simulink model "Drone_simulation_PX4"  (R2025b)
settings: Solver=FixedStepAuto  StartTime=0.0  StopTime=inf  RelTol=1e-6
undefined symbols (not defined in the file): CommParams, fractalcoef, g, Gravity, HIL_GPS_Ts, HIL_HEARTBEAT_Ts, HIL_SENSOR_Ts, HIL_STATE_QUATERNION_Ts, IC, omega_max, Payload, PhysicalScaling, rho_0, SimParams, tau_motor, Tmax_total, Total_mass
libraries: uavmavlinklib x25, slrealtimeiplib x6, sim3dlib x4, aerolibatmos2 x2, matrix_library x1, simulink_extras x1, aerolibasang x1, sensorgpslib x1, mspsensorlib x1, sharedutil x1, aerolibconvert2 x1
(part 1 of 3)
settings Model: Creator=marku  LastModifiedBy=marku
settings SolverCC: AutoInsertRateTranBlk=on
settings OptimizationCC: DefaultParameterBehavior=Inlined  EnhancedBackFolding=on  PassReuseOutputArgsAs=Individual arguments  ZeroExternalMemoryAtStartup=off  ZeroInternalMemoryAtStartup=off  MaxStackSize=64  OptimizeBlockOrder=speed  DifferentSizesBufferReuse=on  OptimizationCustomize=off  EfficientTunableParamExpr=on
settings DebuggingCC: IntegerOverflowMsg=none  ParameterPrecisionLossMsg=none  ParameterTunabilityLossMsg=error  IntegerSaturationMsg=none
settings HardwareCC: ProdBitPerPointer=32.0  ProdBitPerSizeT=32.0  ProdBitPerPtrDiffT=32.0  ProdLargestAtomicInteger=Long  ProdLargestAtomicFloat=Double  ProdWordSize=32.0  ProdHWDeviceType=ARM Compatible->ARM Cortex
settings ModelReferenceCC: EnableParallelModelReferenceBuilds=on
settings SFSimCC: MATLABDynamicMemAlloc=off
settings RTWCC: SystemTargetFile=ert.tlc  TemplateMakefile=ert_default_tmf  Toolchain=GNU Tools for PX4 Autopilots  Description=Embedded Coder
settings CodeAppCC: ForceParamTrailComments=on  IgnoreCustomStorageClasses=off  OperatorAnnotations=on  SimulinkDataObjDesc=on  SFDataObjDesc=on  InsertBlockDesc=on
settings ERTTargetCC: ExtModeTransport=2.0  ExtModeStaticAlloc=on  ExtModeMexFile=ext_xcp  ExtModeIntrfLevel=Level2 - Open  InlinedParameterPlacement=Hierarchical  ERTCustomFileTemplate=example_file_process.tlc  SupportContinuousTime=on

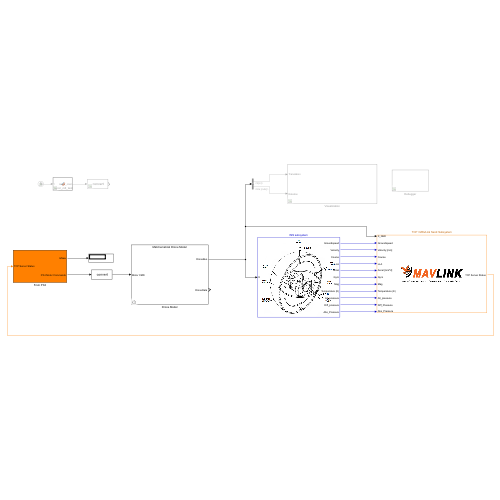
[thumbnail: Simulink's stored preview of the top-level diagram]
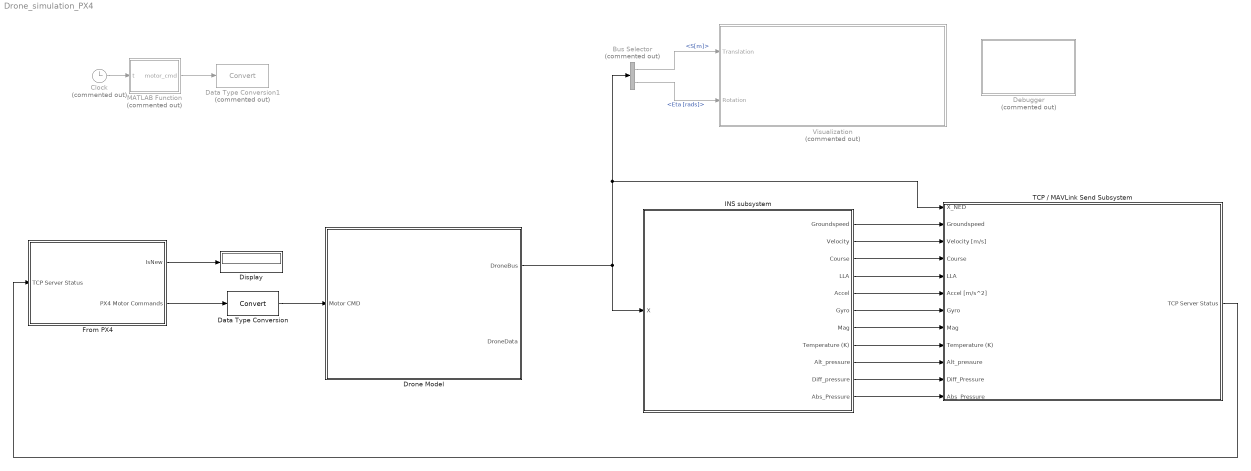
== system Drone_simulation_PX4 ==
  Bus Selector : BusSelector  Commented=on  OutputSignals=State.S[m],State.Eta [rads]
  Clock : Clock  Commented=on
  Data Type Conversion : DataTypeConversion  SaturateOnIntegerOverflow=off  RndMeth=Floor
  Data Type Conversion1 : DataTypeConversion  Commented=on  SaturateOnIntegerOverflow=off  RndMeth=Floor
  Debugger : Subsystem  Commented=on
  Display : Display
  Drone Model : Subsystem  Variant=on
  From PX4 : Subsystem
  INS subsystem : Subsystem
      mask Display: image('INS.png');
  MATLAB Function : MATLAB Function  Commented=on  TreatAsAtomicUnit=on
  TCP / MAVLink Send Subsystem : Subsystem
      mask Display: image('MavLink.png');
  Visualization : Subsystem  Commented=on
  wires:
  INS subsystem/10(Diff_pressure) -> TCP / MAVLink Send Subsystem/11(Diff_Pressure)
  INS subsystem/1(Groundspeed) -> TCP / MAVLink Send Subsystem/2(Groundspeed)
  INS subsystem/2(Velocity) -> TCP / MAVLink Send Subsystem/3(Velocity [m/s])
  INS subsystem/3(Course) -> TCP / MAVLink Send Subsystem/4(Course)
  INS subsystem/4(LLA) -> TCP / MAVLink Send Subsystem/5(LLA)
  INS subsystem/5(Accel) -> TCP / MAVLink Send Subsystem/6(Accel [m/s^2])
  INS subsystem/6(Gyro) -> TCP / MAVLink Send Subsystem/7(Gyro)
  INS subsystem/7(Mag) -> TCP / MAVLink Send Subsystem/8(Mag)
  INS subsystem/8(Temperature (K)) -> TCP / MAVLink Send Subsystem/9(Temperature (K))
  INS subsystem/9(Alt_pressure) -> TCP / MAVLink Send Subsystem/10(Alt_pressure)
  INS subsystem/11(Abs_Pressure) -> TCP / MAVLink Send Subsystem/12(Abs_Pressure)
  TCP / MAVLink Send Subsystem/1(TCP Server Status) -> From PX4/1(TCP Server Status)
  Bus Selector/1 -> Visualization/1(Translation)  "<S[m]>"
  Drone Model/1(DroneBus) -> Bus Selector/1, TCP / MAVLink Send Subsystem/1(X_NED), INS subsystem/1(X)
  Bus Selector/2 -> Visualization/2(Rotation)  "<Eta [rads]>"
  Clock/1 -> MATLAB Function/1(t)
  MATLAB Function/1(motor_cmd) -> Data Type Conversion1/1
  Data Type Conversion/1 -> Drone Model/1(Motor CMD)
  From PX4/2(PX4 Motor Commands) -> Data Type Conversion/1
  From PX4/1(IsNew) -> Display/1

== system Drone_simulation_PX4/Debugger ==
  Bus Creator : BusCreator  Inputs=6
  Clock : Clock
  Constant : Constant  Value=3
  Hover : Constant  Value=-Total_mass*Gravity
  MATLAB Function : MATLAB Function  TreatAsAtomicUnit=on
  MATLAB Function1 : MATLAB Function  TreatAsAtomicUnit=on
  MATLAB Function2 : MATLAB Function  TreatAsAtomicUnit=on
  Manual Switch : ManualSwitch  CurrentSetting=0
  TCP / MAVLink Send Subsystem1 : Subsystem
      mask Display: image('MavLink.png');
  wires:
  MATLAB Function/6(Orientation) -> Bus Creator/6
  MATLAB Function1/1(m) -> Manual Switch/1
  Clock/1 -> MATLAB Function1/1(t)
  MATLAB Function/5(Eta) -> Bus Creator/5
  Hover/1 -> MATLAB Function2/3(T_hover)
  MATLAB Function/2(S_dot) -> Bus Creator/2
  MATLAB Function/1(S) -> Bus Creator/1
  MATLAB Function/4(Omega) -> Bus Creator/4
  Constant/1 -> MATLAB Function1/2(test_id)
  MATLAB Function/3(S_ddot) -> Bus Creator/3

== system Drone_simulation_PX4/Drone Model ==
  Motor CMD : Inport
  Matchematical Drone Model : Subsystem  TreatAsAtomicUnit=on  VariantControl=Config.Plant.VariantValue == 1
  Simscape_Drone_Model : ModelReference  ModelNameDialog=Simscape_Drone_Model.slx  SimulationMode=Normal  VariantControl=Config.Plant.VariantValue == 2  ModelReferenceVersion=1.166
  DroneBus : Outport
  DroneData : Outport  Port=2

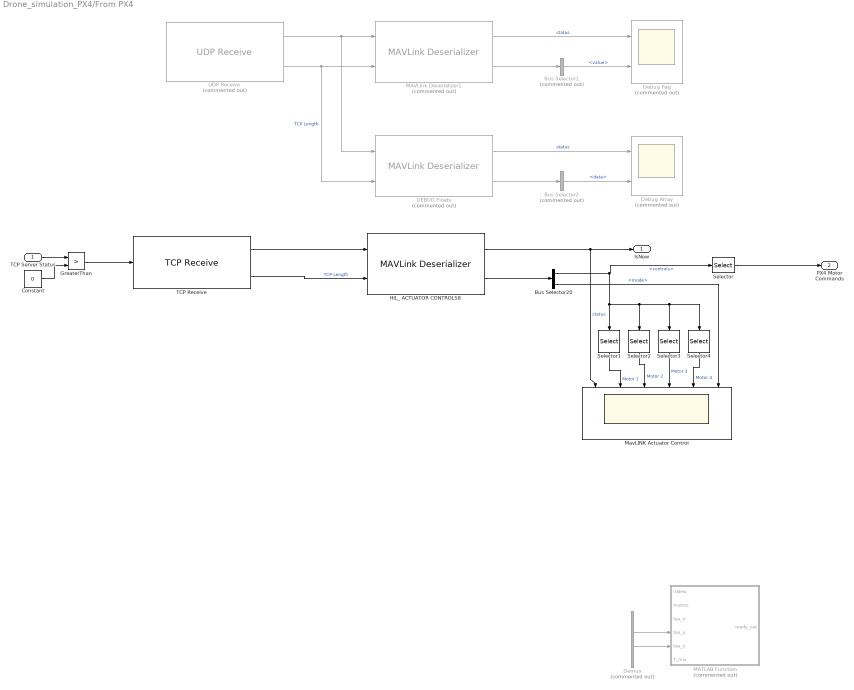
== system Drone_simulation_PX4/From PX4 ==
  TCP Server Status : Inport
  Bus Selector1 : BusSelector  Commented=on  OutputSignals=Payload.value
  Bus Selector2 : BusSelector  Commented=on  OutputSignals=Payload.data
  Bus Selector20 : BusSelector  OutputSignals=Payload.controls,Payload.mode
  Constant : Constant  Value=0  OutDataTypeStr=Inherit: Inherit via back propagation  SampleTime=-1
  DEBUG Floats : uavmavlinklib/MAVLink Deserializer  Commented=on  dialectSource=Select from standard MAVLink dialects  dialect=common.xml  dialectCustom=common.xml  version=2  messageType=DEBUG_FLOAT_ARRAY  inputDataLength=on  SystemIDFilter=off  systemID=1  ComponentIDFilter=off  componentID=1  queueMsg=off  queueMsgSize=50  dropNum=off
  Debug Array : Scope  Commented=on  NumInputPorts=2
      settings: ActiveDisplayYMinimum=-1  ActiveDisplayYMaximum=1  DataLoggingVariableName=ScopeData6
  Debug flag : Scope  Commented=on  NumInputPorts=2
      settings: ActiveDisplayYMinimum=-1  ActiveDisplayYMaximum=1  DataLoggingVariableName=ScopeData9
  Demux : Demux  Commented=on
  GreaterThan : RelationalOperator  Operator=>  OutDataTypeStr=Inherit: Inherit via back propagation  RndMeth=Simplest  InputSameDT=off
  HIL_ ACTUATOR CONTROLS8 : uavmavlinklib/MAVLink Deserializer  dialectSource=Select from standard MAVLink dialects  dialect=common.xml  dialectCustom=common.xml  version=2  messageType=HIL_ACTUATOR_CONTROLS  inputDataLength=on  SystemIDFilter=off  systemID=1  ComponentIDFilter=off  componentID=1  queueMsg=off  queueMsgSize=50  dropNum=off
  MATLAB Function : MATLAB Function  Commented=on  TreatAsAtomicUnit=on
  MAVLink Deserializer1 : uavmavlinklib/MAVLink Deserializer  Commented=on  dialectSource=Select from standard MAVLink dialects  dialect=common.xml  dialectCustom=common.xml  version=2  messageType=DEBUG  inputDataLength=on  SystemIDFilter=off  systemID=1  ComponentIDFilter=off  componentID=1  queueMsg=off  queueMsgSize=50  dropNum=off
  MavLINK Actuator Control : Scope  NumInputPorts=6
      settings: ActiveDisplayYMinimum=-0.12499999999999997  ActiveDisplayYMaximum=1.125  DataLoggingVariableName=ScopeData28
  Selector : Selector  InputPortWidth=16  IndexOptions=Index vector (dialog)  Indices=[1 2 3 4]  OutputSizes=1
  Selector1 : Selector  InputPortWidth=16  IndexOptions=Index vector (dialog)  Indices=[1]  OutputSizes=1
  Selector2 : Selector  InputPortWidth=16  IndexOptions=Index vector (dialog)  Indices=[2]  OutputSizes=1
  Selector3 : Selector  InputPortWidth=16  IndexOptions=Index vector (dialog)  Indices=[3]  OutputSizes=1
  Selector4 : Selector  InputPortWidth=16  IndexOptions=Index vector (dialog)  Indices=[4]  OutputSizes=1
  TCP Receive : slrealtimeiplib/TCP Receive  socketAddPortVal=Server: <Use host-target connection>:4560  rcvWidth=512  sampleTime=-1
  UDP Receive : slrealtimeiplib/UDP Receive  Commented=on  useHostTargetConn=on  ipAddress=0.0.0.0  localPort=14540  rcvWidth=512  rcvFmAny=on  fmAddress='10.10.10.10'  sampleTime=-1  enableMessage=off  maxPackets=1
  IsNew : Outport
  PX4 Motor Commands : Outport  Port=2
  wires:
  Bus Selector2/1 -> Debug Array/2  "<data>"
  HIL_ ACTUATOR CONTROLS8/1 -> MavLINK Actuator Control/1, IsNew/1  "status"
  UDP Receive/2 -> DEBUG Floats/2, MAVLink Deserializer1/2  "TCP Length"
  UDP Receive/1 -> DEBUG Floats/1, MAVLink Deserializer1/1
  Bus Selector20/1 -> Selector/1, Selector2/1, Selector3/1, Selector4/1, Selector1/1  "<controls>"
  Bus Selector1/1 -> Debug flag/2  "<value>"
  Bus Selector20/2 -> MavLINK Actuator Control/6  "<mode>"
  TCP Receive/1 -> HIL_ ACTUATOR CONTROLS8/1
  MAVLink Deserializer1/2 -> Bus Selector1/1
  DEBUG Floats/1 -> Debug Array/1  "status"
  MAVLink Deserializer1/1 -> Debug flag/1  "status"
  TCP Receive/2 -> HIL_ ACTUATOR CONTROLS8/2  "TCP Length"
  HIL_ ACTUATOR CONTROLS8/2 -> Bus Selector20/1
  DEBUG Floats/2 -> Bus Selector2/1
  Selector/1 -> PX4 Motor Commands/1
  TCP Server Status/1 -> GreaterThan/1
  Constant/1 -> GreaterThan/2
  GreaterThan/1 -> TCP Receive/1
  ? -> Demux/1
  Demux/2 -> MATLAB Function/4(tau_y)
  Demux/3 -> MATLAB Function/5(tau_z)
  Selector1/1 -> MavLINK Actuator Control/2  "Motor 1"
  Selector2/1 -> MavLINK Actuator Control/3  "Motor 2"
  Selector3/1 -> MavLINK Actuator Control/4  "Motor 3"
  Selector4/1 -> MavLINK Actuator Control/5  "Motor 4"

== system Drone_simulation_PX4/INS subsystem ==
  X : Inport
  INS : Subsystem
      mask Display: image('INS.png');
  INS Data : Scope  Commented=on  NumInputPorts=11
      settings: ActiveDisplayString=10  ActiveDisplayYMinimum=-1.5003434559985596  ActiveDisplayYMaximum=13.503091103987041  DataLoggingVariableName=ScopeData3
  Groundspeed : Outport
  Velocity : Outport  Port=2
  Course : Outport  Port=3
  LLA : Outport  Port=4
  Accel : Outport  Port=5
  Gyro : Outport  Port=6
  Mag : Outport  Port=7
  Temperature (K) : Outport  Port=8
  Alt_pressure : Outport  Port=9
  Diff_pressure : Outport  Port=10
  Abs_Pressure : Outport  Port=11
  wires:
  INS/3(Groundspeed) -> Groundspeed/1, INS Data/3  "Groundpseed"
  INS/5(Accel) -> Accel/1, INS Data/5  "Acceleration"
  INS/1(LLA) -> LLA/1, INS Data/1  "LLA"
  INS/2(Velocity) -> Velocity/1, INS Data/2  "Velocity"
  INS/4(Course) -> Course/1, INS Data/4  "Course"
  INS/6(Gyro) -> Gyro/1, INS Data/6  "Gyro"
  INS/7(Mag) -> Mag/1, INS Data/7  "Mag"
  INS/8(Temperature (K)) -> Temperature (K)/1, INS Data/8  "Temperature [K]"
  INS/9(Alt_Pressure) -> Alt_pressure/1, INS Data/9  "Alt_pressure"
  INS/10(Diff_Pressure) -> Diff_pressure/1, INS Data/10  "Diff_pressure"
  INS/11(Abs_Pressure) -> Abs_Pressure/1, INS Data/11  "Abs_pressure"
  X/1 -> INS/1(X)

== system Drone_simulation_PX4/TCP // MAVLink Send Subsystem ==
  note: TCP Server
  note: Mavlink
  X_NED : Inport
  Groundspeed : Inport  Port=2
  Velocity [m/s] : Inport  Port=3
  Course : Inport  Port=4
  LLA : Inport  Port=5
  Accel [m/s^2] : Inport  Port=6
  Gyro : Inport  Port=7
  Mag : Inport  Port=8
  Temperature (K) : Inport  Port=9
  Alt_pressure : Inport  Port=10
  Diff_Pressure : Inport  Port=11
  Abs_Pressure : Inport  Port=12
  MAVLink Message Setup : Subsystem
  TCP : Subsystem
  TCP Server Status : Outport
  wires:
  Course/1 -> MAVLink Message Setup/4(Course)
  Groundspeed/1 -> MAVLink Message Setup/2(Groundspeed)
  Velocity [m/s]/1 -> MAVLink Message Setup/3(Velocity [m/s])
  Gyro/1 -> MAVLink Message Setup/7(Gyro)
  MAVLink Message Setup/1(MavLink Message) -> TCP/1(MavLink Message)
  Mag/1 -> MAVLink Message Setup/8(Mag)
  LLA/1 -> MAVLink Message Setup/5(LLA)
  Temperature (K)/1 -> MAVLink Message Setup/9(Temperature (K))
  Accel [m/s^2]/1 -> MAVLink Message Setup/6(Accel [m/s^2])
  Alt_pressure/1 -> MAVLink Message Setup/10(Alt_pressure)
  Diff_Pressure/1 -> MAVLink Message Setup/11(Diff_Pressure)
  X_NED/1 -> MAVLink Message Setup/1(X_NED)
  Abs_Pressure/1 -> MAVLink Message Setup/12(Abs_Pressure)
  TCP/1(TCP Server Status) -> TCP Server Status/1

== system Drone_simulation_PX4/Visualization ==
  Translation : Inport
  Rotation : Inport  Port=2
  Camera : sim3dlib/Simulation 3D Actor  Priority=1  ActorName=Sim3dActor2  ParentName=Scene Origin  Operation=Create at setup  InitScriptText=|  SampleTime=-1  Translation=[0 0 0]  Rotation=[0 0 0]  Scale=[1 1 1]  InputsText=Sim3dActor2.Translation Sim3dActor2.Rotation  aMode=5  ActorTag=Sim3dActor2  ActorType=Sim3dActor  ID=2
      | % Reserved keywords:
      | % - Actor : handle to this actor object
      | % - World : handle to the world object
      | 
      | % Examples:
      | 
      | % Create a primitive geometry (optional)
      | % createShape(Actor, 'box', [1 1 1]);
      | 
      | % Initialize values (optional)
      | % Actor.Physics = true;
      | % Actor.Color = [1 0 0];
  Constant : Constant  Value=[0; 0; 0]
  Gain : Gain  Gain=[-1; -1; 1]
  Simulation 3D Actor : sim3dlib/Simulation 3D Actor  Priority=1  ActorName=Sim3dActor1  ParentName=Scene Origin  Operation=Create at setup  InitScriptText=|  SampleTime=-1  Translation=[0 0 0]  Rotation=[0 0 0]  Scale=[1 1 1]  InputsText=Sim3dActor1.Translation Sim3dActor1.Rotation  aMode=5  ActorTag=Sim3dActor1  ActorType=Sim3dActor  ID=1
      | % Generic body shape for the 3D view (unit drone: 0.5 m across the rotors).
      | createShape(Actor, 'box', [0.5 0.5 0.1]);
  Simulation 3D Scene Configuration : sim3dlib/Simulation 3D Scene Configuration  Priority=0  ProjectFormat=Default Scenes  SceneDesc=Open surface  ProjectName=C:\Program Files\MATLAB\R2025b\toolbox\shared\sim3d_projects\automotive_project_windows\UE\WindowsNoEditor\VehicleSimulation.exe  ScenePath=/Game/Maps/HwStrght  EnableOpenDRIVE=off  vehTagList={'Custom';'Scene Origin';'Sim3dActor1';'Sim3dActor2'}  vehTag=Sim3dActor2  AttachedCameraRelativeTranslation=[-3 -3 2]  FreeCameraDefaultInitialTranslation=[-6, 0, 2]  AttachedCameraRelativeRotation=[-0 -20 45]  FreeCameraDefaultInitialRotation=[0, -15, 0]  ViewpointName=Custom  FreeCameraInitialTranslation=[-4 -4 2]  ViewpointTranslation=[0 0 0]  FreeCameraInitialRotation=[0 -15 45]  ViewpointRotation=[0 0 0]  OpVisEn=off  Ts=0.02  EnableWindow=off  EnableRemoteAccess=off  EnableWeather=off  SunAzimuth=90  SunAltitude=40.0  EnableGeospatialSun=off  Latitude=0  Longitude=0  Date=2023-01-01  Time=10:30:00  GeoTimeZone=-5.0  SunDaylightSaving=off  wind=1  clouds=10  EnableVolumetricClouds=off  CloudCoverage=0  CloudAltitude=6  fog=0  rain=0  RaindropsEffect=off  SnowDensity=0  EnableGeospatial=off  TilesetSource=Earth terrain  UseTrueOrigin=off  OriginHeight=200  OriginLatitude=40.744652  OriginLongitude=-73.988864  MapStyle=Aerial  AdditionalAssetIDs=[]  UseAdvancedSunSky=off  SolarTime=11  TimeZone=-5  Day=21  Month=9  Year=2022  UseDaylightSavingTime=on  DSTStartDay=10  DSTStartMonth=3  DSTEndDay=3  DSTEndMonth=11  DSTSwitchHour=2  sensorTag=MainCamera1  sensorId=1  sensorName=MainCamera1  mountLoc=Origin  offsetFlag=off  tmountOffset=[0, 0, 0]  rmountOffset=[0, 0, 0]  HorizontalResolution=1280  VerticalResolution=720  HorizontalFOV=60  mountPoint=[0 0 0]  mountOrientation=[0 0 0]  aMode=0  ID=1  GeoTrigger=Inactive  ViewNameList={'Custom'}  ViewTranslationList={'[-4 -4 2]'}  ViewRotationList={'[0 -15 45]'}
      settings: LibrarySourceBlock=aerolibsim3d/Simulation 3D Scene Configuration
  Simulation 3D Video Writer : sim3dlib/Simulation 3D Video Writer  Priority=1  Commented=on  Filename=PX4_square_flight.mp4  FileAction=Overwrite  Interval=[0 inf]  aMode=5
      settings: LibrarySourceBlock=sl3dlib/Simulation 3D/Utilities/Simulation 3D Video Writer
  Terminator : Terminator
  Terminator1 : Terminator
  Transpose : Math  Operator=transpose
  Transpose1 : Math  Operator=transpose
  Transpose2 : Math  Operator=transpose
  wires:
  Transpose/1 -> Camera/1, Simulation 3D Actor/1
  Simulation 3D Actor/1 -> Terminator/1
  Translation/1 -> Transpose/1
  Transpose1/1 -> Simulation 3D Actor/2
  Rotation/1 -> Gain/1
  Constant/1 -> Transpose2/1
  Transpose2/1 -> Camera/2
  Camera/1 -> Terminator1/1
  Gain/1 -> Transpose1/1

== system Drone_simulation_PX4/Debugger/TCP // MAVLink Send Subsystem1 ==
  note: MAVLink Message Setup
  note: TCP Server
  note: Mavlink
  note: Collected Signals
  note: MavLink signal setup
  HIL HEARTBEAT : Subsystem
  HIL STATE QUATERNION : Subsystem  Commented=on
  HIL_GPS : Subsystem
  HIL_SENSOR : Subsystem
  MAVLink Concatenate : Concatenate  NumInputs=4
  Signal Debugging : Subsystem
  TCP : Subsystem
  TCP Server Status : Outport
  wires:
  [A4] -> MAVLink Concatenate/4
  HIL HEARTBEAT/1(HEARTBEAT_DATA) -> [A4]
  [A3] -> MAVLink Concatenate/2
  [A2] -> MAVLink Concatenate/3
  [A1] -> MAVLink Concatenate/1
  MAVLink Concatenate/1 -> TCP/1(MavLink Message)  "MavLink Message"
  HIL STATE QUATERNION/1(HIL_STATE_QUATERNION_bytes) -> [A3], Signal Debugging/1(HIL_STATE_QUATERNION_bytes)
  HIL_SENSOR/1(HIL_SENSOR_bytes) -> Signal Debugging/3(HIL_SENSOR_bytes), [A1]
  HIL_GPS/1(HIL_SENSOR_bytes) -> Signal Debugging/2(HIL_GPS_bytes), [A2]
  TCP/1(TCP Server Status) -> TCP Server Status/1

== system Drone_simulation_PX4/Drone Model/Matchematical Drone Model ==
  Motor CMD : Inport
  Constant : Constant  Value=0
  Drone Dynamics : Subsystem
      mask Display: disp('Mechanical System')
  ENU to NED : Subsystem
      mask Display: image('World Frame Conversion.png');
  Hover : Constant  Commented=on  Value=single(sqrt(Total_mass*g/Tmax_total) * ones(4,1))
  MATLAB Function3 : MATLAB Function  Commented=on  TreatAsAtomicUnit=on
  Out Bus Element1 : Outport  PortName=DroneData  Element=Data
  Out Bus Element : Outport  Port=2  PortName=DroneBus  Element=State
  wires:
  Hover/1 -> MATLAB Function3/3(u_hover_cmd)
  Drone Dynamics/1(Drone_ENU) -> ENU to NED/1(Drone_ENU)
  Constant/1 -> Out Bus Element1/1
  ENU to NED/1(X_NED) -> Out Bus Element/1
  Motor CMD/1 -> Drone Dynamics/1(Inputs), MATLAB Function3/2(m_px4)

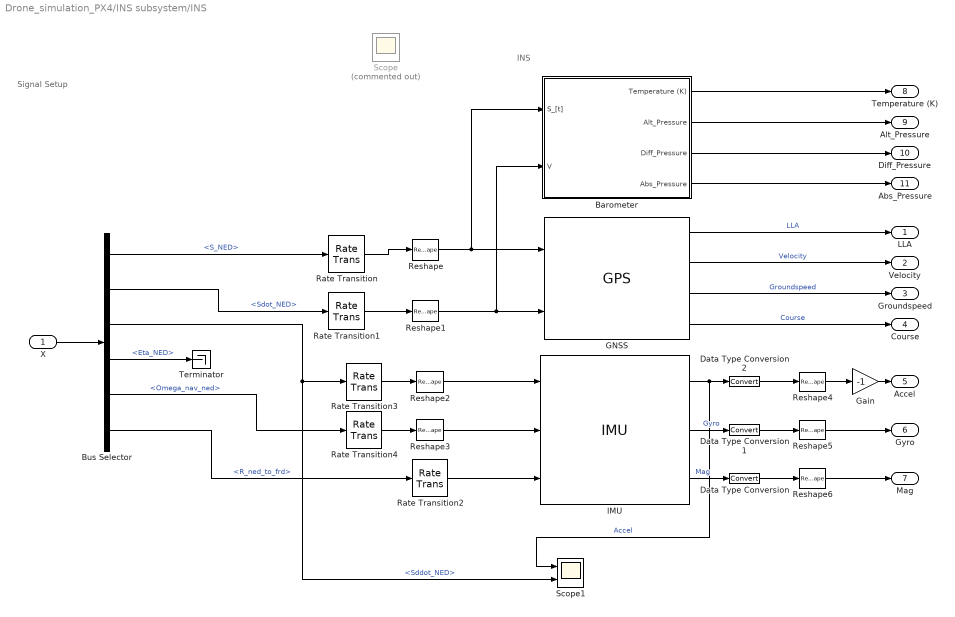
== system Drone_simulation_PX4/INS subsystem/INS ==
  note: INS
  note: Signal Setup
  X : Inport
  Barometer : Subsystem
  Bus Selector : BusSelector  OutputSignals=State.S_NED,State.Sdot_NED,State.Sddot_NED,State.Eta_NED,State.Omega_nav_ned,State.R_ned_to_frd
  Data Type Conversion : DataTypeConversion  SaturateOnIntegerOverflow=off  RndMeth=Floor
  Data Type Conversion1 : DataTypeConversion  SaturateOnIntegerOverflow=off  RndMeth=Floor
  Data Type Conversion2 : DataTypeConversion  SaturateOnIntegerOverflow=off  RndMeth=Floor
  GNSS : sensorgpslib/GPS  DispRefFrame=NED  PositionInputFormat=Local  ReferenceLocation=SimParams.HomeLLA  HorizontalPositionAccuracy=0.001  VerticalPositionAccuracy=0.001  VelocityAccuracy=0.001  DecayFactor=0  SeedDouble=0  SimulateUsing=Code generation
      settings: LibrarySourceBlock=mspsensorlib/GPS
  Gain : Gain  Gain=-1  OutDataTypeStr=Inherit: Inherit via back propagation
  IMU : mspsensorlib/IMU  DispRefFrame=NED  TemperaturePort=off  Temperature=15  MagneticFieldPort=off  MagneticFieldNED=SimParams.MagneticFieldNED  MagneticFieldENU=[ -2.4169, 27.5550, 16.0849 ]  SeedDouble=0  SimulateUsing=Code generation  AccelParamsMeasurementRange=Inf  AccelParamsResolution=0  AccelParamsConstantBias=[ 0, 0, 0 ]  AccelParamsAxesMisalignment=[ 100, 0, 0; 0, 100, 0; 0, 0, 100 ]  AccelParamsNoiseDensity=[ 0, 0, 0 ]  AccelParamsBiasInstability=[ 0, 0, 0 ]  AccelParamsBiasInstabilityNumerator=fractalcoef().Numerator  AccelParamsBiasInstabilityDenominator=fractalcoef().Denominator  AccelParamsRandomWalk=[ 0, 0, 0 ]  AccelParamsNoiseType=double-sided  AccelParamsTemperatureBias=[ 0, 0, 0 ]  AccelParamsTemperatureScaleFactor=[ 0, 0, 0 ]  GyroParamsMeasurementRange=Inf  GyroParamsResolution=0  GyroParamsConstantBias=[ 0, 0, 0 ]  GyroParamsAxesMisalignment=[ 100, 0, 0; 0, 100, 0; 0, 0, 100 ]  GyroParamsAccelerationBias=[ 0, 0, 0 ]  GyroParamsNoiseDensity=[ 0, 0, 0 ]  GyroParamsBiasInstability=[ 0, 0, 0 ]  GyroParamsBiasInstabilityNumerator=fractalcoef().Numerator  GyroParamsBiasInstabilityDenominator=fractalcoef().Denominator  GyroParamsRandomWalk=[ 0, 0, 0 ]  GyroParamsNoiseType=double-sided  GyroParamsTemperatureBias=[ 0, 0, 0 ]  GyroParamsTemperatureScaleFactor=[ 0, 0, 0 ]  MagParamsMeasurementRange=Inf  MagParamsResolution=0  MagParamsConstantBias=[ 0, 0, 0 ]  MagParamsAxesMisalignment=[ 100, 0, 0; 0, 100, 0; 0, 0, 100 ]  MagParamsNoiseDensity=[ 0, 0, 0 ]  MagParamsBiasInstability=[ 0, 0, 0 ]  MagParamsBiasInstabilityNumerator=fractalcoef().Numerator  MagParamsBiasInstabilityDenominator=fractalcoef().Denominator  MagParamsRandomWalk=[ 0, 0, 0 ]  MagParamsNoiseType=double-sided  MagParamsTemperatureBias=[ 0, 0, 0 ]  MagParamsTemperatureScaleFactor=[ 0, 0, 0 ]
  Rate Transition{,1..4} (5 alike) : RateTransition  OutPortSampleTime=CommParams.INS.Ts
  Reshape : Reshape  OutputDimensionality=Customize  OutputDimensions=[1,3]
  Reshape1 : Reshape  OutputDimensionality=Customize  OutputDimensions=[1,3]
  Reshape2 : Reshape  OutputDimensionality=Row vector (2-D)
  Reshape3 : Reshape  OutputDimensionality=Row vector (2-D)
  Reshape4 : Reshape
  Reshape5 : Reshape
  Reshape6 : Reshape
  Scope : Scope  Commented=on
      settings: ActiveDisplayYMinimum=-1  ActiveDisplayYMaximum=1  DataLoggingVariableName=ScopeData10
  Scope1 : Scope  NumInputPorts=2
      settings: ActiveDisplayYMinimum=-8.196879445424031  ActiveDisplayYMaximum=18.133560919726278  DataLoggingVariableName=ScopeData15
  Terminator : Terminator
  LLA : Outport
  Velocity : Outport  Port=2
  Groundspeed : Outport  Port=3
  Course : Outport  Port=4
  Accel : Outport  Port=5
  Gyro : Outport  Port=6
  Mag : Outport  Port=7
  Temperature (K) : Outport  Port=8
  Alt_Pressure : Outport  Port=9
  Diff_Pressure : Outport  Port=10
  Abs_Pressure : Outport  Port=11
  wires:
  GNSS/4 -> Course/1  "Course"
  GNSS/1 -> LLA/1  "LLA"
  GNSS/2 -> Velocity/1  "Velocity"
  GNSS/3 -> Groundspeed/1  "Groundspeed"
  Rate Transition2/1 -> IMU/3
  IMU/2 -> Data Type Conversion1/1  "Gyro"
  IMU/3 -> Data Type Conversion/1  "Mag"
  Rate Transition/1 -> Reshape/1
  Rate Transition1/1 -> Reshape1/1
  Rate Transition3/1 -> Reshape2/1
  Rate Transition4/1 -> Reshape3/1
  Barometer/1(Temperature (K)) -> Temperature (K)/1
  Barometer/2(Alt_Pressure) -> Alt_Pressure/1
  Barometer/3(Diff_Pressure) -> Diff_Pressure/1
  Barometer/4(Abs_Pressure) -> Abs_Pressure/1
  IMU/1 -> Scope1/1, Data Type Conversion2/1  "Accel"
  Reshape4/1 -> Gain/1
  Reshape5/1 -> Gyro/1
  Reshape6/1 -> Mag/1
  Data Type Conversion/1 -> Reshape6/1
  Data Type Conversion1/1 -> Reshape5/1
  Data Type Conversion2/1 -> Reshape4/1
  Gain/1 -> Accel/1
  X/1 -> Bus Selector/1
  Bus Selector/1 -> Rate Transition/1  "<S_NED>"
  Bus Selector/2 -> Rate Transition1/1  "<Sdot_NED>"
  Bus Selector/3 -> Rate Transition3/1, Scope1/2  "<Sddot_NED>"
  Bus Selector/4 -> Terminator/1  "<Eta_NED>"
  Bus Selector/6 -> Rate Transition2/1  "<R_ned_to_frd>"
  Reshape/1 -> Barometer/1(S_[t]), GNSS/1
  Reshape1/1 -> Barometer/2(V), GNSS/2
  Reshape2/1 -> IMU/1
  Reshape3/1 -> IMU/2
  Bus Selector/5 -> Rate Transition4/1  "<Omega_nav_ned>"

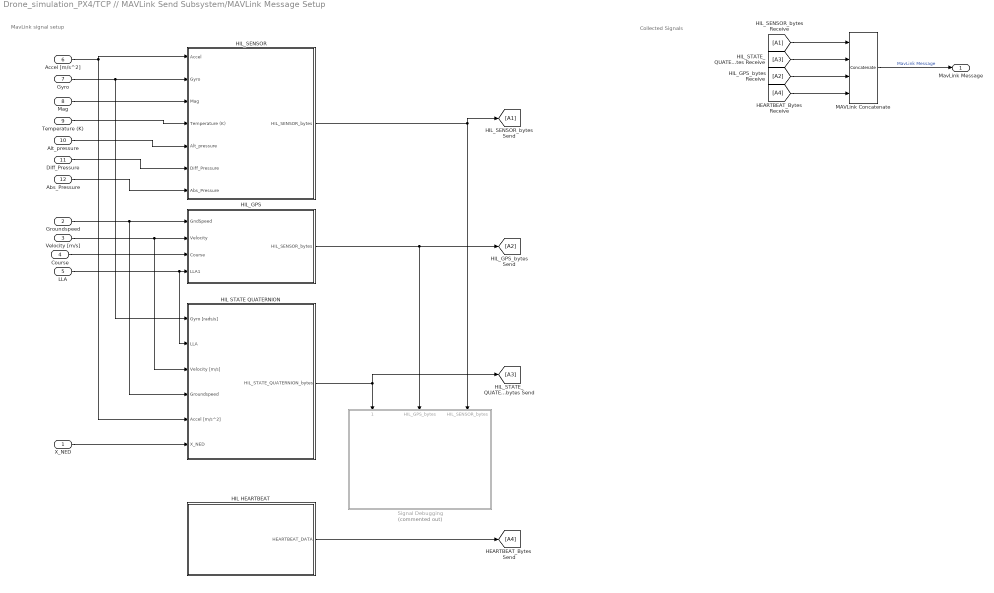
== system Drone_simulation_PX4/TCP // MAVLink Send Subsystem/MAVLink Message Setup ==
  note: MavLink signal setup
  note: Collected Signals
  X_NED : Inport
  Groundspeed : Inport  Port=2
  Velocity [m/s] : Inport  Port=3
  Course : Inport  Port=4
  LLA : Inport  Port=5
  Accel [m/s^2] : Inport  Port=6
  Gyro : Inport  Port=7
  Mag : Inport  Port=8
  Temperature (K) : Inport  Port=9
  Alt_pressure : Inport  Port=10
  Diff_Pressure : Inport  Port=11
  Abs_Pressure : Inport  Port=12
  HIL HEARTBEAT : Subsystem
  HIL STATE QUATERNION : Subsystem
  HIL_GPS : Subsystem
  HIL_SENSOR : Subsystem
  MAVLink Concatenate : Concatenate  NumInputs=4
  Signal Debugging : Subsystem  Commented=on
  MavLink Message : Outport
  wires:
  Alt_pressure/1 -> HIL_SENSOR/5(Alt_pressure)
  Mag/1 -> HIL_SENSOR/3(Mag)
  Diff_Pressure/1 -> HIL_SENSOR/6(Diff_Pressure)
  Temperature (K)/1 -> HIL_SENSOR/4(Temperature (K))
  Gyro/1 -> HIL STATE QUATERNION/1(Gyro [rads/s]), HIL_SENSOR/2(Gyro)
  HIL_GPS/1(HIL_SENSOR_bytes) -> Signal Debugging/2(HIL_GPS_bytes), [A2]
  Accel [m/s^2]/1 -> HIL STATE QUATERNION/5(Accel [m/s^2]), HIL_SENSOR/1(Accel)
  Abs_Pressure/1 -> HIL_SENSOR/7(Abs_Pressure)
  Course/1 -> HIL_GPS/3(Course)
  Velocity [m/s]/1 -> HIL STATE QUATERNION/3(Velocity [m/s]), HIL_GPS/2(Velocity)
  Groundspeed/1 -> HIL STATE QUATERNION/4(Groundspeed), HIL_GPS/1(GndSpeed)
  LLA/1 -> HIL STATE QUATERNION/2(LLA), HIL_GPS/4(LLA1)
  X_NED/1 -> HIL STATE QUATERNION/6(X_NED)
  HIL_SENSOR/1(HIL_SENSOR_bytes) -> Signal Debugging/3(HIL_SENSOR_bytes), [A1]
  HIL STATE QUATERNION/1(HIL_STATE_QUATERNION_bytes) -> [A3], Signal Debugging/1(HIL_STATE_QUATERNION_bytes)
  MAVLink Concatenate/1 -> MavLink Message/1  "MavLink Message"
  [A1] -> MAVLink Concatenate/1
  [A2] -> MAVLink Concatenate/3
  [A3] -> MAVLink Concatenate/2
  HIL HEARTBEAT/1(HEARTBEAT_DATA) -> [A4]
  [A4] -> MAVLink Concatenate/4

== system Drone_simulation_PX4/TCP // MAVLink Send Subsystem/TCP ==
  note: Server setup
  MavLink Message : Inport
  Boolean : Constant  OutDataTypeStr=Inherit: Inherit via back propagation  SampleTime=-1
  Display2 : Display
  Display3 : Display
  Reshape : Reshape
  TCP Send : slrealtimeiplib/TCP Send  socketAddPortVal=Server: <Use host-target connection>:4560  sampleTime=CommParams.HIL.Ts
  TCP Server : slrealtimeiplib/TCP Server  Priority=-1  useHostTargetConn=on  serverAddress=172.29.112.1  serverPort=4560  useNaglesAlgorithm=on
  Width : Width
  TCP Server Status : Outport
  wires:
  MavLink Message/1 -> Reshape/1
  TCP Server/1 -> TCP Server Status/1, Display2/1
  Boolean/1 -> TCP Server/1, TCP Send/1
  Reshape/1 -> TCP Send/2, Width/1
  TCP Send/1 -> Display3/1
  Width/1 -> TCP Send/3

== system Drone_simulation_PX4/Debugger/TCP // MAVLink Send Subsystem1/HIL HEARTBEAT ==
  Bus Assignment : BusAssignment  AssignedSignals=Payload.custom_mode,Payload.type,Payload.autopilot,Payload.base_mode,Payload.system_status,Payload.mavlink_version
  Constant : Constant  Value=0  OutDataTypeStr=Inherit: Inherit via back propagation  SampleTime=HIL_HEARTBEAT_Ts
  Constant1 : Constant  Value=2  OutDataTypeStr=Inherit: Inherit via back propagation  SampleTime=HIL_HEARTBEAT_Ts
  Constant2 : Constant  Value=8  OutDataTypeStr=Inherit: Inherit via back propagation  SampleTime=HIL_HEARTBEAT_Ts
  Constant3 : Constant  Value=0  OutDataTypeStr=Inherit: Inherit via back propagation  SampleTime=HIL_HEARTBEAT_Ts
  Constant4 : Constant  Value=4  OutDataTypeStr=Inherit: Inherit via back propagation  SampleTime=HIL_HEARTBEAT_Ts
  Constant5 : Constant  Value=3  OutDataTypeStr=Inherit: Inherit via back propagation  SampleTime=HIL_HEARTBEAT_Ts
  MAVLink Blank Message : uavmavlinklib/MAVLink Blank Message  dialectSource=Select from standard MAVLink dialects  dialect=common.xml  dialectCustom=common.xml  version=2  messageType=HEARTBEAT  SystemID=2  ComponentID=51  SampleTime=HIL_HEARTBEAT_Ts
  MAVLink Serializer : uavmavlinklib/MAVLink Serializer  dialectSource=Select from standard MAVLink dialects  dialect=common.xml  dialectCustom=common.xml  version=2  messageType=HEARTBEAT
  Rate Transition : RateTransition  OutPortSampleTime=HIL_HEARTBEAT_Ts
  Terminator : Terminator
  HEARTBEAT_DATA : Outport
  wires:
  Constant4/1 -> Bus Assignment/6
  Constant2/1 -> Bus Assignment/4
  MAVLink Blank Message/1 -> Bus Assignment/1
  Constant3/1 -> Bus Assignment/5
  Constant1/1 -> Bus Assignment/3
  Constant/1 -> Bus Assignment/2
  Constant5/1 -> Bus Assignment/7
  Bus Assignment/1 -> Rate Transition/1
  Rate Transition/1 -> MAVLink Serializer/1
  MAVLink Serializer/1 -> HEARTBEAT_DATA/1
  MAVLink Serializer/2 -> Terminator/1

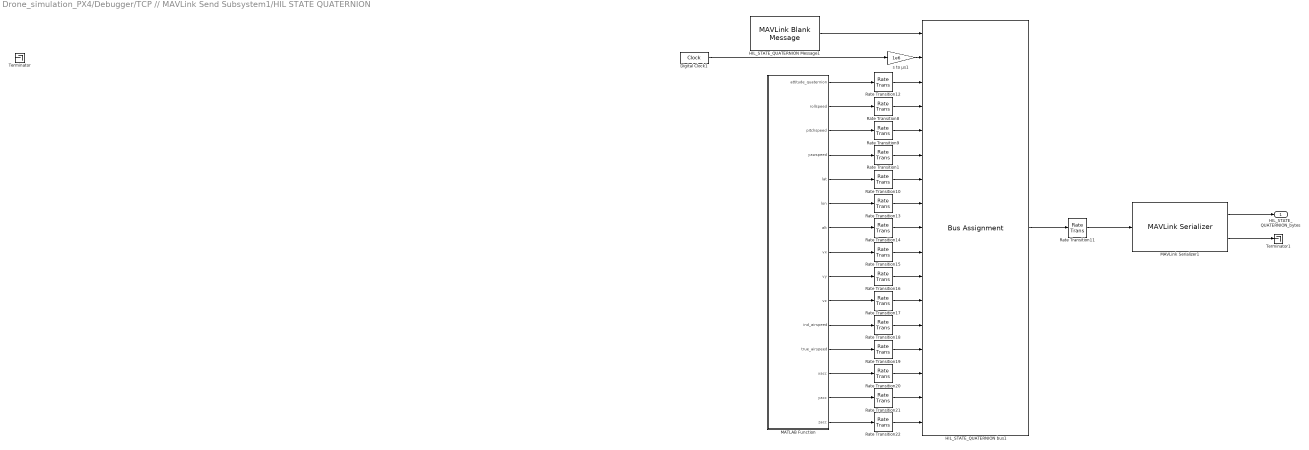
== system Drone_simulation_PX4/Debugger/TCP // MAVLink Send Subsystem1/HIL STATE QUATERNION ==
  Digital Clock1 : DigitalClock  SampleTime=HIL_STATE_QUATERNION_Ts
  HIL_STATE_QUATERNION Message1 : uavmavlinklib/MAVLink Blank Message  dialectSource=Select from standard MAVLink dialects  dialect=common.xml  dialectCustom=common.xml  version=2  messageType=HIL_STATE_QUATERNION  SystemID=2  ComponentID=51  SampleTime=-1
  HIL_STATE_QUATERNION bus1 : BusAssignment  AssignedSignals=Payload.time_usec,Payload.attitude_quaternion,Payload.rollspeed,Payload.pitchspeed,Payload.yawspeed,Payload.lat,Payload.lon,Payload.alt,Payload.vx,Payload.vy,Payload.vz,Payload.ind_airspeed,Payload.true_airspeed,Payload.xacc,Payload.yacc,Payload.zacc
  MATLAB Function : MATLAB Function  TreatAsAtomicUnit=on
  MAVLink Serializer1 : uavmavlinklib/MAVLink Serializer  dialectSource=Select from standard MAVLink dialects  dialect=common.xml  dialectCustom=common.xml  version=2  messageType=HIL_STATE_QUATERNION
  Rate Transition{1,8..22} (16 alike) : RateTransition  OutPortSampleTime=HIL_STATE_QUATERNION_Ts
  Terminator : Terminator
  Terminator1 : Terminator
  s to µs1 : Gain  Gain=1e6  OutDataTypeStr=uint64
  HIL_STATE_QUATERNION_bytes : Outport
  wires:
  Rate Transition11/1 -> MAVLink Serializer1/1
  HIL_STATE_QUATERNION bus1/1 -> Rate Transition11/1
  MAVLink Serializer1/2 -> Terminator1/1
  MAVLink Serializer1/1 -> HIL_STATE_QUATERNION_bytes/1
  HIL_STATE_QUATERNION Message1/1 -> HIL_STATE_QUATERNION bus1/1
  s to µs1/1 -> HIL_STATE_QUATERNION bus1/2
  Digital Clock1/1 -> s to µs1/1
  Rate Transition22/1 -> HIL_STATE_QUATERNION bus1/17
  Rate Transition21/1 -> HIL_STATE_QUATERNION bus1/16
  Rate Transition20/1 -> HIL_STATE_QUATERNION bus1/15
  Rate Transition19/1 -> HIL_STATE_QUATERNION bus1/14
  Rate Transition18/1 -> HIL_STATE_QUATERNION bus1/13
  Rate Transition12/1 -> HIL_STATE_QUATERNION bus1/3
  Rate Transition8/1 -> HIL_STATE_QUATERNION bus1/4
  Rate Transition9/1 -> HIL_STATE_QUATERNION bus1/5
  Rate Transition1/1 -> HIL_STATE_QUATERNION bus1/6
  Rate Transition10/1 -> HIL_STATE_QUATERNION bus1/7
  Rate Transition13/1 -> HIL_STATE_QUATERNION bus1/8
  Rate Transition14/1 -> HIL_STATE_QUATERNION bus1/9
  Rate Transition15/1 -> HIL_STATE_QUATERNION bus1/10
  Rate Transition16/1 -> HIL_STATE_QUATERNION bus1/11
  Rate Transition17/1 -> HIL_STATE_QUATERNION bus1/12
  MATLAB Function/1(attitude_quaternion) -> Rate Transition12/1
  MATLAB Function/2(rollspeed) -> Rate Transition8/1
  MATLAB Function/3(pitchspeed) -> Rate Transition9/1
  MATLAB Function/4(yawspeed) -> Rate Transition1/1
  MATLAB Function/5(lat) -> Rate Transition10/1
  MATLAB Function/6(lon) -> Rate Transition13/1
  MATLAB Function/7(alt) -> Rate Transition14/1
  MATLAB Function/8(vx) -> Rate Transition15/1
  MATLAB Function/9(vy) -> Rate Transition16/1
  MATLAB Function/10(vz) -> Rate Transition17/1
  MATLAB Function/11(ind_airspeed) -> Rate Transition18/1
  MATLAB Function/12(true_airspeed) -> Rate Transition19/1
  MATLAB Function/13(xacc) -> Rate Transition20/1
  MATLAB Function/14(yacc) -> Rate Transition21/1
  MATLAB Function/15(zacc) -> Rate Transition22/1

== system Drone_simulation_PX4/Debugger/TCP // MAVLink Send Subsystem1/HIL_GPS ==
  Digital Clock : DigitalClock  SampleTime=HIL_GPS_Ts
  HIL_GPS Bus : BusAssignment  AssignedSignals=Payload.time_usec,Payload.lat,Payload.lon,Payload.alt,Payload.eph,Payload.epv,Payload.vel,Payload.vn,Payload.ve,Payload.vd,Payload.cog,Payload.fix_type,Payload.satellites_visible
  HIL_GPS Message : uavmavlinklib/MAVLink Blank Message  dialectSource=Select from standard MAVLink dialects  dialect=common.xml  dialectCustom=common.xml  version=2  messageType=HIL_GPS  SystemID=2  ComponentID=51  SampleTime=HIL_GPS_Ts
  MATLAB Function : MATLAB Function  TreatAsAtomicUnit=on
  MAVLink Serializer : uavmavlinklib/MAVLink Serializer  dialectSource=Select from standard MAVLink dialects  dialect=common.xml  dialectCustom=common.xml  version=2  messageType=HIL_GPS
  Rate Transition{,1..12} (13 alike) : RateTransition  OutPortSampleTime=HIL_GPS_Ts
  Terminator : Terminator
  s to µs : Gain  Gain=1e6  OutDataTypeStr=uint64
  HIL_SENSOR_bytes : Outport
  wires:
  Rate Transition/1 -> MAVLink Serializer/1
  HIL_GPS Message/1 -> HIL_GPS Bus/1
  s to µs/1 -> HIL_GPS Bus/2
  HIL_GPS Bus/1 -> Rate Transition/1
  Digital Clock/1 -> s to µs/1
  MAVLink Serializer/2 -> Terminator/1
  MAVLink Serializer/1 -> HIL_SENSOR_bytes/1
  MATLAB Function/1(lat) -> Rate Transition5/1
  MATLAB Function/2(lon) -> Rate Transition1/1
  MATLAB Function/3(alt) -> Rate Transition3/1
  MATLAB Function/4(eph) -> Rate Transition2/1
  MATLAB Function/5(epv) -> Rate Transition8/1
  MATLAB Function/6(vel) -> Rate Transition4/1
  MATLAB Function/7(vn) -> Rate Transition7/1
  MATLAB Function/8(ve) -> Rate Transition6/1
  MATLAB Function/9(vd) -> Rate Transition12/1
  MATLAB Function/10(cog) -> Rate Transition9/1
  MATLAB Function/11(fix_type) -> Rate Transition11/1
  MATLAB Function/12(satellites_visible) -> Rate Transition10/1
  Rate Transition5/1 -> HIL_GPS Bus/3
  Rate Transition1/1 -> HIL_GPS Bus/4
  Rate Transition2/1 -> HIL_GPS Bus/6
  Rate Transition3/1 -> HIL_GPS Bus/5
  Rate Transition6/1 -> HIL_GPS Bus/10
  Rate Transition8/1 -> HIL_GPS Bus/7
  Rate Transition7/1 -> HIL_GPS Bus/9
  Rate Transition4/1 -> HIL_GPS Bus/8
  Rate Transition12/1 -> HIL_GPS Bus/11
  Rate Transition10/1 -> HIL_GPS Bus/14
  Rate Transition11/1 -> HIL_GPS Bus/13
  Rate Transition9/1 -> HIL_GPS Bus/12

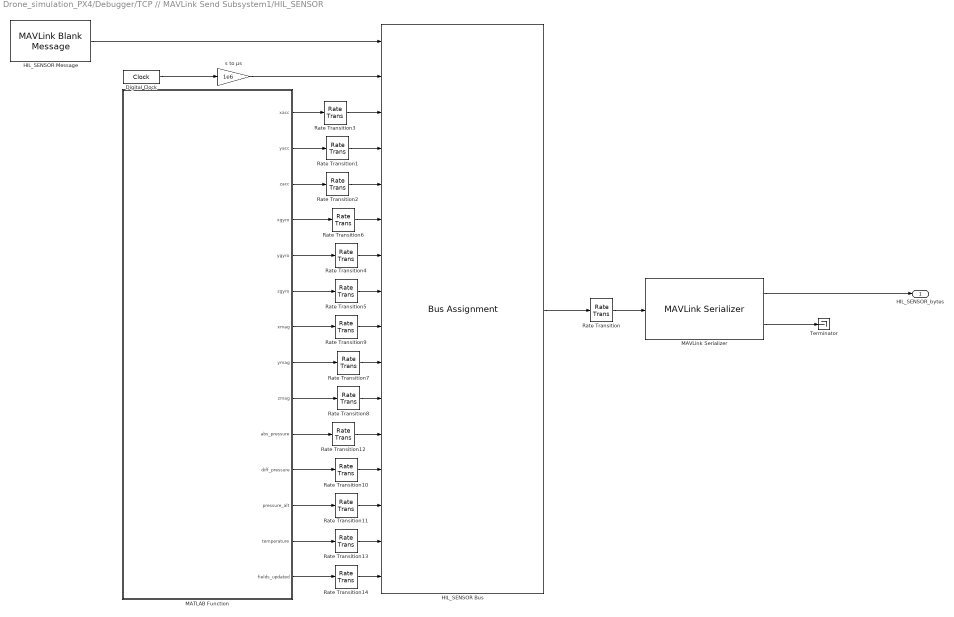
== system Drone_simulation_PX4/Debugger/TCP // MAVLink Send Subsystem1/HIL_SENSOR ==
  Digital Clock : DigitalClock  SampleTime=HIL_SENSOR_Ts
  HIL_SENSOR Bus : BusAssignment  AssignedSignals=Payload.time_usec,Payload.xacc,Payload.yacc,Payload.zacc,Payload.xgyro,Payload.ygyro,Payload.zgyro,Payload.xmag,Payload.ymag,Payload.zmag,Payload.abs_pressure,Payload.diff_pressure,Payload.pressure_alt,Payload.temperature,Payload.fields_updated
  HIL_SENSOR Message : uavmavlinklib/MAVLink Blank Message  dialectSource=Select from standard MAVLink dialects  dialect=common.xml  dialectCustom=common.xml  version=2  messageType=HIL_SENSOR  SystemID=2  ComponentID=51  SampleTime=HIL_SENSOR_Ts
  MATLAB Function : MATLAB Function  TreatAsAtomicUnit=on
  MAVLink Serializer : uavmavlinklib/MAVLink Serializer  dialectSource=Select from standard MAVLink dialects  dialect=common.xml  dialectCustom=common.xml  version=2  messageType=HIL_SENSOR
  Rate Transition{,1..14} (15 alike) : RateTransition  OutPortSampleTime=HIL_SENSOR_Ts
  Terminator : Terminator
  s to µs : Gain  Gain=1e6  OutDataTypeStr=uint64
  HIL_SENSOR_bytes : Outport
  wires:
  Rate Transition/1 -> MAVLink Serializer/1
  HIL_SENSOR Message/1 -> HIL_SENSOR Bus/1
  HIL_SENSOR Bus/1 -> Rate Transition/1
  Digital Clock/1 -> s to µs/1
  s to µs/1 -> HIL_SENSOR Bus/2
  MAVLink Serializer/2 -> Terminator/1
  MAVLink Serializer/1 -> HIL_SENSOR_bytes/1
  MATLAB Function/1(xacc) -> Rate Transition3/1
  MATLAB Function/2(yacc) -> Rate Transition1/1
  MATLAB Function/3(zacc) -> Rate Transition2/1
  MATLAB Function/4(xgyro) -> Rate Transition6/1
  MATLAB Function/5(ygyro) -> Rate Transition4/1
  MATLAB Function/6(zgyro) -> Rate Transition5/1
  MATLAB Function/7(xmag) -> Rate Transition9/1
  MATLAB Function/8(ymag) -> Rate Transition7/1
  MATLAB Function/9(zmag) -> Rate Transition8/1
  MATLAB Function/10(abs_pressure) -> Rate Transition12/1
  MATLAB Function/11(diff_pressure) -> Rate Transition10/1
  MATLAB Function/12(pressure_alt) -> Rate Transition11/1
  MATLAB Function/13(temperature) -> Rate Transition13/1
  MATLAB Function/14(fields_updated) -> Rate Transition14/1
  Rate Transition3/1 -> HIL_SENSOR Bus/3
  Rate Transition1/1 -> HIL_SENSOR Bus/4
  Rate Transition2/1 -> HIL_SENSOR Bus/5
  Rate Transition5/1 -> HIL_SENSOR Bus/8
  Rate Transition6/1 -> HIL_SENSOR Bus/6
  Rate Transition4/1 -> HIL_SENSOR Bus/7
  Rate Transition8/1 -> HIL_SENSOR Bus/11
  Rate Transition9/1 -> HIL_SENSOR Bus/9
  Rate Transition7/1 -> HIL_SENSOR Bus/10
  Rate Transition12/1 -> HIL_SENSOR Bus/12
  Rate Transition10/1 -> HIL_SENSOR Bus/13
  Rate Transition11/1 -> HIL_SENSOR Bus/14
  Rate Transition14/1 -> HIL_SENSOR Bus/16
  Rate Transition13/1 -> HIL_SENSOR Bus/15

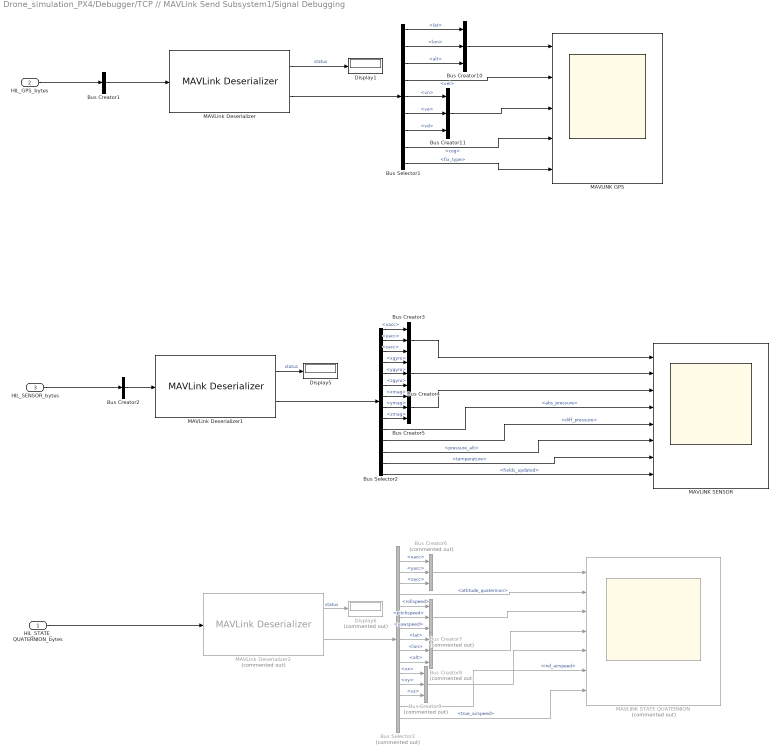
== system Drone_simulation_PX4/Debugger/TCP // MAVLink Send Subsystem1/Signal Debugging ==
  HIL_STATE_QUATERNION_bytes : Inport
  HIL_GPS_bytes : Inport  Port=2
  HIL_SENSOR_bytes : Inport  Port=3
  Bus Creator1 : BusCreator  Inputs=1
  Bus Creator{3..5,10..11} (5 alike) : BusCreator  Inputs=3
  Bus Creator2 : BusCreator  Inputs=1
  Bus Creator{6..9} (4 alike) : BusCreator  Commented=on  Inputs=3
  Bus Selector1 : BusSelector  OutputSignals=Payload.lat,Payload.lon,Payload.alt,Payload.vel,Payload.vn,Payload.ve,Payload.vd,Payload.cog,Payload.fix_type
  Bus Selector2 : BusSelector  OutputSignals=Payload.xacc,Payload.yacc,Payload.zacc,Payload.xgyro,Payload.ygyro,Payload.zgyro,Payload.xmag,Payload.ymag,Payload.zmag,Payload.abs_pressure,Payload.diff_pressure,Payload.pressure_alt,Payload.temperature,Payload.fields_updated
  Bus Selector3 : BusSelector  Commented=on  OutputSignals=Payload.xacc,Payload.yacc,Payload.zacc,Payload.attitude_quaternion,Payload.rollspeed,Payload.pitchspeed,Payload.yawspeed,Payload.lat,Payload.lon,Payload.alt,Payload.vx,Payload.vy,Payload.vz,Payload.ind_airspeed,Payload.true_airspeed
  Display1 : Display
  Display5 : Display
  Display6 : Display  Commented=on
  MAVLINK GPS : Scope  NumInputPorts=5
      settings: ActiveDisplayYMinimum=-1  ActiveDisplayYMaximum=1
  MAVLINK SENSOR : Scope  NumInputPorts=8
      settings: ActiveDisplayYMinimum=-1  ActiveDisplayYMaximum=1
  MAVLINK STATE QUATERNION : Scope  Commented=on  NumInputPorts=7
      settings: ActiveDisplayYMinimum=-0.088388346135616289  ActiveDisplayYMaximum=0.79549511522054672
  MAVLink Deserializer : uavmavlinklib/MAVLink Deserializer  dialectSource=Select from standard MAVLink dialects  dialect=common.xml  dialectCustom=common.xml  version=2  messageType=HIL_GPS  inputDataLength=off  SystemIDFilter=off  systemID=1  ComponentIDFilter=off  componentID=1  queueMsg=off  queueMsgSize=50  dropNum=off
  MAVLink Deserializer1 : uavmavlinklib/MAVLink Deserializer  dialectSource=Select from standard MAVLink dialects  dialect=common.xml  dialectCustom=common.xml  version=2  messageType=HIL_SENSOR  inputDataLength=off  SystemIDFilter=off  systemID=1  ComponentIDFilter=off  componentID=1  queueMsg=off  queueMsgSize=50  dropNum=off
  MAVLink Deserializer2 : uavmavlinklib/MAVLink Deserializer  Commented=on  dialectSource=Select from standard MAVLink dialects  dialect=common.xml  dialectCustom=common.xml  version=2  messageType=HIL_STATE_QUATERNION  inputDataLength=off  SystemIDFilter=off  systemID=1  ComponentIDFilter=off  componentID=1  queueMsg=off  queueMsgSize=50  dropNum=off
  wires:
  Bus Selector2/10 -> MAVLINK SENSOR/4  "<abs_pressure>"
  Bus Creator1/1 -> MAVLink Deserializer/1
  Bus Selector2/3 -> Bus Creator3/3  "<zacc>"
  Bus Selector1/9 -> MAVLINK GPS/5  "<fix_type>"
  Bus Selector2/4 -> Bus Creator4/1  "<xgyro>"
  Bus Selector2/7 -> Bus Creator5/1  "<xmag>"
  Bus Selector2/6 -> Bus Creator4/3  "<zgyro>"
  MAVLink Deserializer1/1 -> Display5/1  "status"
  Bus Selector1/4 -> MAVLINK GPS/2  "<vel>"
  Bus Selector2/9 -> Bus Creator5/3  "<zmag>"
  Bus Selector1/8 -> MAVLINK GPS/4  "<cog>"
  Bus Selector2/12 -> MAVLINK SENSOR/6  "<pressure_alt>"
  Bus Selector2/11 -> MAVLINK SENSOR/5  "<diff_pressure>"
  MAVLink Deserializer/1 -> Display1/1  "status"
  Bus Selector2/8 -> Bus Creator5/2  "<ymag>"
  Bus Creator3/1 -> MAVLINK SENSOR/1
  Bus Creator4/1 -> MAVLINK SENSOR/2
  MAVLink Deserializer/2 -> Bus Selector1/1
  Bus Creator2/1 -> MAVLink Deserializer1/1
  MAVLink Deserializer1/2 -> Bus Selector2/1
  Bus Creator5/1 -> MAVLINK SENSOR/3
  Bus Selector2/1 -> Bus Creator3/1  "<xacc>"
  Bus Selector2/13 -> MAVLINK SENSOR/7  "<temperature>"
  HIL_GPS_bytes/1 -> Bus Creator1/1
  Bus Selector2/14 -> MAVLINK SENSOR/8  "<fields_updated>"
  Bus Selector2/2 -> Bus Creator3/2  "<yacc>"
  Bus Selector2/5 -> Bus Creator4/2  "<ygyro>"
  HIL_SENSOR_bytes/1 -> Bus Creator2/1
  HIL_STATE_QUATERNION_bytes/1 -> MAVLink Deserializer2/1
  MAVLink Deserializer2/2 -> Bus Selector3/1
  MAVLink Deserializer2/1 -> Display6/1  "status"
  Bus Selector3/1 -> Bus Creator6/1  "<xacc>"
  Bus Selector3/2 -> Bus Creator6/2  "<yacc>"
  Bus Selector3/3 -> Bus Creator6/3  "<zacc>"
  Bus Selector3/5 -> Bus Creator7/1  "<rollspeed>"
  Bus Selector3/6 -> Bus Creator7/2  "<pitchspeed>"
  Bus Selector3/7 -> Bus Creator7/3  "<yawspeed>"
  Bus Selector3/8 -> Bus Creator8/1  "<lat>"
  Bus Selector3/9 -> Bus Creator8/2  "<lon>"
  Bus Selector3/10 -> Bus Creator8/3  "<alt>"
  Bus Selector3/11 -> Bus Creator9/1  "<vx>"
  Bus Selector3/12 -> Bus Creator9/2  "<vy>"
  Bus Selector3/13 -> Bus Creator9/3  "<vz>"
  Bus Selector3/14 -> MAVLINK STATE QUATERNION/6  "<ind_airspeed>"
  Bus Selector3/15 -> MAVLINK STATE QUATERNION/7  "<true_airspeed>"
  Bus Creator6/1 -> MAVLINK STATE QUATERNION/1
  Bus Selector3/4 -> MAVLINK STATE QUATERNION/2  "<attitude_quaternion>"
  Bus Creator7/1 -> MAVLINK STATE QUATERNION/3
  Bus Creator8/1 -> MAVLINK STATE QUATERNION/4
  Bus Creator9/1 -> MAVLINK STATE QUATERNION/5
  Bus Selector1/1 -> Bus Creator10/1  "<lat>"
  Bus Selector1/2 -> Bus Creator10/2  "<lon>"
  Bus Selector1/3 -> Bus Creator10/3  "<alt>"
  Bus Selector1/7 -> Bus Creator11/3  "<vd>"
  Bus Selector1/6 -> Bus Creator11/2  "<ve>"
  Bus Selector1/5 -> Bus Creator11/1  "<vn>"
  Bus Creator11/1 -> MAVLINK GPS/3
  Bus Creator10/1 -> MAVLINK GPS/1

== system Drone_simulation_PX4/Debugger/TCP // MAVLink Send Subsystem1/TCP ==
  note: Server setup
  MavLink Message : Inport
  Boolean : Constant  OutDataTypeStr=Inherit: Inherit via back propagation  SampleTime=-1
  Display2 : Display
  Display3 : Display
  Reshape : Reshape
  TCP Send : slrealtimeiplib/TCP Send  socketAddPortVal=Server: <Use host-target connection>:4560  sampleTime=0.004
  TCP Server : slrealtimeiplib/TCP Server  Priority=-1  useHostTargetConn=on  serverAddress=0.0.0.0  serverPort=4560  useNaglesAlgorithm=on
  Width : Width
  TCP Server Status : Outport
  wires:
  MavLink Message/1 -> Reshape/1
  TCP Server/1 -> TCP Server Status/1, Display2/1
  Boolean/1 -> TCP Server/1, TCP Send/1
  Reshape/1 -> TCP Send/2, Width/1
  TCP Send/1 -> Display3/1
  Width/1 -> TCP Send/3

== system Drone_simulation_PX4/Drone Model/Matchematical Drone Model/Drone Dynamics ==
  Inputs : Inport
  Bus Creator1 : BusCreator  Inputs=6
  Bus Selector : BusSelector  OutputSignals=Thrust,Torques
  MATLAB Function : MATLAB Function  Commented=on  TreatAsAtomicUnit=on
  Mechnical System : Subsystem
      settings: PortSchema="{\"entries\":[{\"content\":{\"sides\":[{\"content\":{\"connectorIds\":[\"In1\"]},\"type\":\"ConnectorPlacement.EquallySpacedRectSide\",\"uuid\":\"e23cf896-6c75-4ce8-966c-2c3fb68d880b\"},{\"content\":{\"connectorIds\":[\"Out1\",\"Out2\",\"Out3\",\"Out4\",\"Out5\",\"Out6\"],\"side\":\"RIGHT\"},\"type\":\"ConnectorPlacement.EquallySpacedRectSide\",\"uuid\":\"331013fa-80da-45af-80bf-25ac247d6e9d\"},{\"content\":{\"side\":\"TOP\"},\"type\":\"ConnectorPlacement.EquallySpacedRectSide\",\"uuid\":\"91f65d57-cc6c-4d1e-bf12-791766af4195\"},{\"content\":{\"connectorIds\":[\"Out7\",\"Out8\"],\"side\":\"BOTTOM\"},\"type\":\"ConnectorPlacement.EquallySpacedRectSide\",\"uuid\":\"5a15da3c-47de-44ae-815a-d356ead639d1\"}]},\"type\":\"ConnectorPlacement.EquallySpacedConnector\",\"uuid\":\"93f2c743-5085-41e0-beba-771e8ac9e4c3\"}],\"packageUris\":[\"http://schema.mathworks.com/mf0/Connector/R2020b\"],\"version\":\"1.0\"}"
  Motor Rotor System : Subsystem
      settings: PortSchema="{\"entries\":[{\"content\":{\"sides\":[{\"content\":{\"connectorIds\":[\"In1\"]},\"type\":\"ConnectorPlacement.EquallySpacedRectSide\",\"uuid\":\"403d2ce0-86ef-4d72-9184-ea93c232084b\"},{\"content\":{\"connectorIds\":[\"Out1\"],\"side\":\"RIGHT\"},\"type\":\"ConnectorPlacement.EquallySpacedRectSide\",\"uuid\":\"c9f820ca-b75b-463f-bf2d-4f8ba610756b\"},{\"content\":{\"side\":\"TOP\"},\"type\":\"ConnectorPlacement.EquallySpacedRectSide\",\"uuid\":\"6f1167bf-b926-47ec-8f0c-f121015de8c9\"},{\"content\":{\"connectorIds\":[\"In2\"],\"side\":\"BOTTOM\"},\"type\":\"ConnectorPlacement.EquallySpacedRectSide\",\"uuid\":\"c077359a-e737-4c99-b474-8284cf89f3c1\"}]},\"type\":\"ConnectorPlacement.EquallySpacedConnector\",\"uuid\":\"2d6bb495-36aa-4654-a5a9-b40a367231e7\"}],\"packageUris\":[\"http://schema.mathworks.com/mf0/Connector/R2020b\"],\"version\":\"1.0\"}"
  Radians to Degrees : simulink_extras/Transformations/Radians to Degrees
  True Data (ENU) : Scope  NumInputPorts=7
      settings: ActiveDisplayString=6  ActiveDisplayYMinimum=-0.0070755809800233374  ActiveDisplayYMaximum=0.0082880225344592884  DataLoggingVariableName=ScopeData5
  Drone_ENU : Outport
  wires:
  Mechnical System/2(S_dot [m/s]) -> True Data (ENU)/2, Bus Creator1/2  "S_dot [m/s]"
  Bus Selector/1 -> True Data (ENU)/5  "<Thrust>"
  Mechnical System/1(S [m]) -> True Data (ENU)/1, Bus Creator1/1  "S [m]"
  Bus Selector/2 -> True Data (ENU)/6  "<Torques>"
  Mechnical System/5(Eta [Rads]) -> Radians to Degrees/1, Bus Creator1/5  "Eta [rads]"
  Mechnical System/4(Omega [rads/s]) -> Bus Creator1/4, True Data (ENU)/7
  Bus Creator1/1 -> Drone_ENU/1
  Mechnical System/3(S_ddot [m/s^2]) -> Bus Creator1/3, True Data (ENU)/3  "S_ddot [m/s^2]"
  Mechnical System/6(Orientation) -> Bus Creator1/6
  Mechnical System/8(Drone inputs) -> Bus Selector/1
  Inputs/1 -> Motor Rotor System/1(Motor CMD)
  Mechnical System/7(Rho) -> Motor Rotor System/2(Rho)
  Radians to Degrees/1 -> True Data (ENU)/4  "Eta [degrees]"
  Motor Rotor System/1(Drone inputs) -> Mechnical System/1(Torques and Thurst)

== system Drone_simulation_PX4/Drone Model/Matchematical Drone Model/ENU to NED ==
  Drone_ENU : Inport
  Bus Selector : BusSelector  OutputSignals=S [m],S_dot [m/s],S_ddot [m/s^2],Omega [rads/s],Eta [rads],Orientation
  MATLAB Function : MATLAB Function  TreatAsAtomicUnit=on
  S_ENU : Scope  Commented=on  NumInputPorts=6
      settings: ActiveDisplayString=6  ActiveDisplayYMinimum=-1  ActiveDisplayYMaximum=1  DataLoggingVariableName=ScopeData12
  S_NED : Scope  NumInputPorts=6
      settings: ActiveDisplayString=6  ActiveDisplayYMinimum=-1.25  ActiveDisplayYMaximum=1.25  DataLoggingVariableName=ScopeData8
  Terminator1 : Terminator
  Terminator2 : Terminator
  X_ned : BusCreator  Inputs=6
  X_NED : Outport
  wires:
  Drone_ENU/1 -> Bus Selector/1
  MATLAB Function/2(Sdot_ned) -> S_NED/2, X_ned/2  "Sdot_NED"
  MATLAB Function/1(S_ned) -> X_ned/1, S_NED/1  "S_NED"
  MATLAB Function/6(Eta_ned) -> S_NED/5, X_ned/4  "Eta_NED"
  MATLAB Function/3(Sddot_ned) -> X_ned/3, S_NED/3  "Sddot_NED"
  X_ned/1 -> X_NED/1  "X_NED"
  Bus Selector/1 -> S_ENU/1, MATLAB Function/1(S_enu)  "<S [m]>"
  Bus Selector/2 -> MATLAB Function/2(Sdot_enu)  "<S_dot [m/s]>"
  Bus Selector/3 -> MATLAB Function/3(Sddot_enu)  "<S_ddot [m/s^2]>"
  Bus Selector/4 -> MATLAB Function/4(Omega_flu)  "<Omega [rads/s]>"
  Bus Selector/5 -> MATLAB Function/5(Eta_enu)  "<Eta [rads]>"
  Bus Selector/6 -> MATLAB Function/6(R_enu)  "<Orientation>"
  MATLAB Function/5(Omega_nav_ned) -> S_NED/4, X_ned/5  "Omega_nav_ned"
  MATLAB Function/8(R_ned_to_frd) -> S_NED/6, X_ned/6
  MATLAB Function/7(R_ned) -> Terminator1/1  "R_ned"
  MATLAB Function/4(Omega_frd) -> Terminator2/1  "Omega_NED"

== system Drone_simulation_PX4/INS subsystem/INS/Barometer ==
  S_[t] : Inport
  V : Inport  Port=2
  Dynamic Pressure : aerolibasang/Dynamic Pressure
  Gain : Gain  Gain=-1
  ISA Atmosphere Model : aerolibatmos2/ISA Atmosphere Model  useExtended=off  action=None  custom=off  viscosityOut=off  g=9.80665  gamma=1.4  R=287.0531  L=0.0065  h_trop=11000  h_strat=20000  rho0=1.225  P0=101325  T0=288.15  h0=0  S=110.4  Tref=273.15  muref=1.716e-5
  Pressure Altitude : aerolibatmos2/Pressure Altitude  units=Metric (MKS)  action=Warning
  Selector4 : Selector  InputPortWidth=3  IndexOptions=Index vector (dialog)  Indices=[3]  OutputSizes=1
  Terminator : Terminator
  Temperature (K) : Outport
  Alt_Pressure : Outport  Port=2
  Diff_Pressure : Outport  Port=3
  Abs_Pressure : Outport  Port=4
  wires:
  ISA Atmosphere Model/1 -> Temperature (K)/1
  ISA Atmosphere Model/4 -> Dynamic Pressure/2
  Selector4/1 -> Gain/1  "Z_ned"
  ISA Atmosphere Model/3 -> Abs_Pressure/1, Pressure Altitude/1
  S_[t]/1 -> Selector4/1
  Pressure Altitude/1 -> Alt_Pressure/1
  Dynamic Pressure/1 -> Diff_Pressure/1
  ISA Atmosphere Model/2 -> Terminator/1
  V/1 -> Dynamic Pressure/1
  Gain/1 -> ISA Atmosphere Model/1
